simulink model "simuidentJose1"  (R2020a)
settings: Solver=VariableStepAuto  StartTime=0.0  StopTime=24  RelTol=1e-3
values from neighbouring files (symbols this model uses):
  Cc = pidtune(G, 'PIDF', opt)    [identManuel.m]
  vetorDenominadorG = rand(1, size(G.Denominator, 2))    [identJose.m]
  vetorNumeradorG = rand(1, size(G.Numerator,2))    [identJose.m]
  yMaximo = 6    [identJose.m]
libraries: simulink x3
settings Model: EnablePacing=on  PacingRate=1000  Creator=eduma  LastModifiedBy=eduma
settings DataIOCC: InspectSignalLogs=on

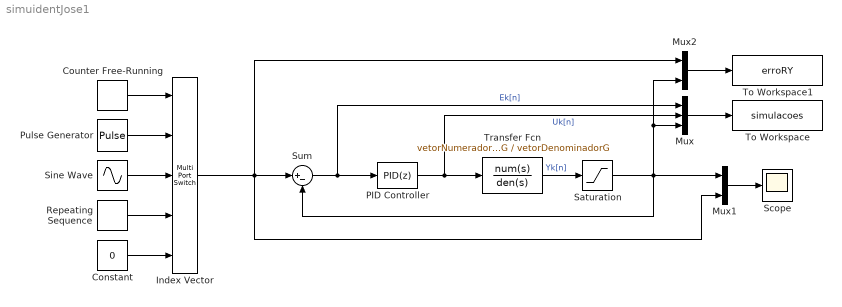
== system simuidentJose1 ==
  Constant : Constant  Value=0
  Counter Free-Running : simulink/Sources/Counter Free-Running  NumBits=24  tsamp=8
  Index Vector : MultiPortSwitch  DataPortOrder=Zero-based contiguous  DataPortForDefault=Additional data port  DiagnosticForDefault=None  zeroidx=on
  Mux : Mux  Inputs=3
  Mux1 : Mux  Inputs=2
  Mux2 : Mux  Inputs=2
  PID Controller : simulink/Continuous/PID Controller  Controller=PID  Form=Parallel  TimeDomain=Discrete-time  UseExternalTs=off  SampleTime=2/1000  IntegratorMethod=Forward Euler  FilterMethod=Forward Euler  ControllerParametersSource=internal  P=Cc.Kp  I=Cc.Ki  D=Cc.Kd  UseFilter=on  N=1 / Cc.Tf  TunerSelectOption=Transfer Function Based (PID Tuner App)  InitialConditionSource=internal  InitialConditionForIntegrator=0  InitialConditionForFilter=0  DifferentiatorICPrevScaledInput=0  ExternalReset=none  TrackingMode=off  Kt=1  LimitOutput=on  UpperSaturationLimit=1  LowerSaturationLimit=0  LinearizeAsGain=off  AntiWindupMode=none  Kb=1  POutMin=[]  POutMax=[]  IOutMin=[]  IOutMax=[]  DOutMin=[]  DOutMax=[]  NOutMin=[]  NOutMax=[]  SumOutMin=[]  SumOutMax=[]  SaturationOutMin=[]  SaturationOutMax=[]  PParamMin=[]  PParamMax=[]  IParamMin=[]  IParamMax=[]  DParamMin=[]  DParamMax=[]  NParamMin=[]  NParamMax=[]  KbParamMin=[]  KbParamMax=[]  KtParamMin=[]  KtParamMax=[]  KbOutMin=[]  KbOutMax=[]  KtOutMin=[]  KtOutMax=[]  IntegratorOutMin=[]  IntegratorOutMax=[]  FilterOutMin=[]  FilterOutMax=[]  SumI1OutMin=[]  SumI1OutMax=[]  SumI2OutMin=[]  SumI2OutMax=[]  SumI3OutMin=[]  SumI3OutMax=[]  SumI4OutMin=[]  SumI4OutMax=[]  SumDOutMin=[]  SumDOutMax=[]  DifferentiatorOutMin=[]  DifferentiatorOutMax=[]  FilterDiffOutCoefMin=[]  FilterDiffOutCoefMax=[]  ReciprocalOutMin=[]  ReciprocalOutMax=[]  SumDenOutMin=[]  SumDenOutMax=[]  SumNumOutMin=[]  SumNumOutMax=[]  DivideOutMin=[]  DivideOutMax=[]  UdiffTsProdOutMin=[]  UdiffTsProdOutMax=[]  NTsProdOutMin=[]  NTsProdOutMax=[]  UintegralTsProdOutMin=[]  UintegralTsProdOutMax=[]  UngainTsProdOutMin=[]  UngainTsProdOutMax=[]  IntegratorContinuousStateAttributes=''  IntegratorStateMustResolveToSignalObject=off  IntegratorRTWStateStorageClass=Auto  FilterContinuousStateAttributes=''  FilterStateMustResolveToSignalObject=off  FilterRTWStateStorageClass=Auto  ParallelPVariant=InternalParameters  IdealPVariant=Disabled  IVariant=InternalParameters  DVariant=InternalParameters  IntegratorVariant=Discrete  SatVariant=Enabled  AWVariant=Passthrough  PCopyVariant=Disabled  TRVariant=Disabled  FdbkBlocksVariant=Forward  IdealPFdbkVariant=Disabled  SatFdbkVariant=Disabled  DerivativeFilterVariant=ForwardEulerFilter  NVariant=InternalParameters  NCopyVariant=Disabled  FilterICVariant=InternalICsFilter  IntegratorICVariant=InternalICs  ExternalResetVariant=Disabled  TRSumVariant=Passthrough  SumFdbkVariant=Disabled  SumVariant=Sum_PID  TsampFilterVariant=InternalTs  TsampNgainVariant=Passthrough  TsampIntegralVariant=Passthrough
  Pulse Generator : DiscretePulseGenerator  PulseType=Time based  Amplitude=yMaximo  Period=8  PulseWidth=50  PhaseDelay=4
  Repeating Sequence : simulink/Sources/Repeating Sequence  rep_seq_t=[0 2 4]  rep_seq_y=[0 yMaximo 0]
  Saturation : Saturate  UpperLimit=40  LowerLimit=-10
  Scope : Scope
  Sine Wave : Sin  Amplitude=yMaximo / 2  Bias=yMaximo / 2  SampleTime=0
  Sum : Sum  Inputs=|+-
  To Workspace : ToWorkspace  VariableName=simulacoes  SaveFormat=Timeseries  SampleTime=-1
  To Workspace1 : ToWorkspace  VariableName=erroRY  SaveFormat=Timeseries  SampleTime=-1
  Transfer Fcn : TransferFcn  Numerator=vetorNumeradorG  Denominator=vetorDenominadorG  AbsoluteTolerance=1000
  wires:
  PID Controller/1 -> Mux/2, Transfer Fcn/1  "Uk[n]"
  Sum/1 -> Mux/1, PID Controller/1  "Ek[n]"
  Mux/1 -> To Workspace/1
  Counter Free-Running/1 -> Index Vector/1
  Repeating Sequence/1 -> Index Vector/4
  Sine Wave/1 -> Index Vector/3
  Pulse Generator/1 -> Index Vector/2
  Mux1/1 -> Scope/1
  Constant/1 -> Index Vector/5
  Index Vector/1 -> Mux1/2, Mux2/1, Sum/1
  Mux2/1 -> To Workspace1/1
  Transfer Fcn/1 -> Saturation/1  "Yk[n]"
  Saturation/1 -> Sum/2, Mux2/2, Mux/3, Mux1/1
